simulink model "OnlyCurrent"  (R2025b)
settings: Solver=VariableStepAuto  StartTime=0.0  StopTime=0.3  MaxStep=1/20e3/100  RelTol=1e-3
InitFcn:
  | fs = 20e3;
  | Ts = 1/fs;
  | I2B = 10;
  | UB = 20;
  | freq0 = 50;
  | freqc = 5;
  | w0 = 2*pi / (1/freq0);
  | wc = 2*pi / (1/freqc);
  | I2_Kp = 3.023;
  | I2_Kr = 16.36;
  | UDC = 48;
  | Ic_Kd = 11.55;
libraries: ee_lib x26, nesl_utility x21, fl_lib x18, simulink x1
settings Model: Creator=GoodUser  LastModifiedBy=GoodUser

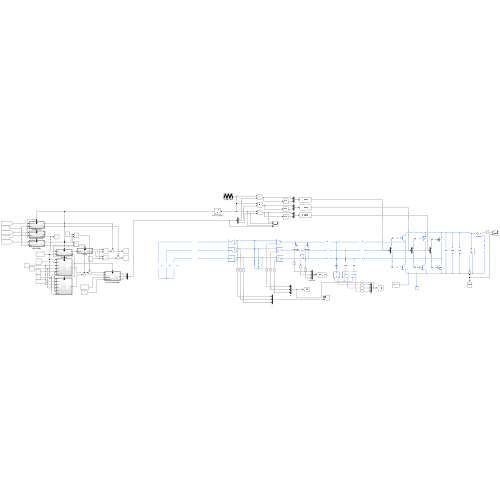
[thumbnail: Simulink's stored preview of the top-level diagram]
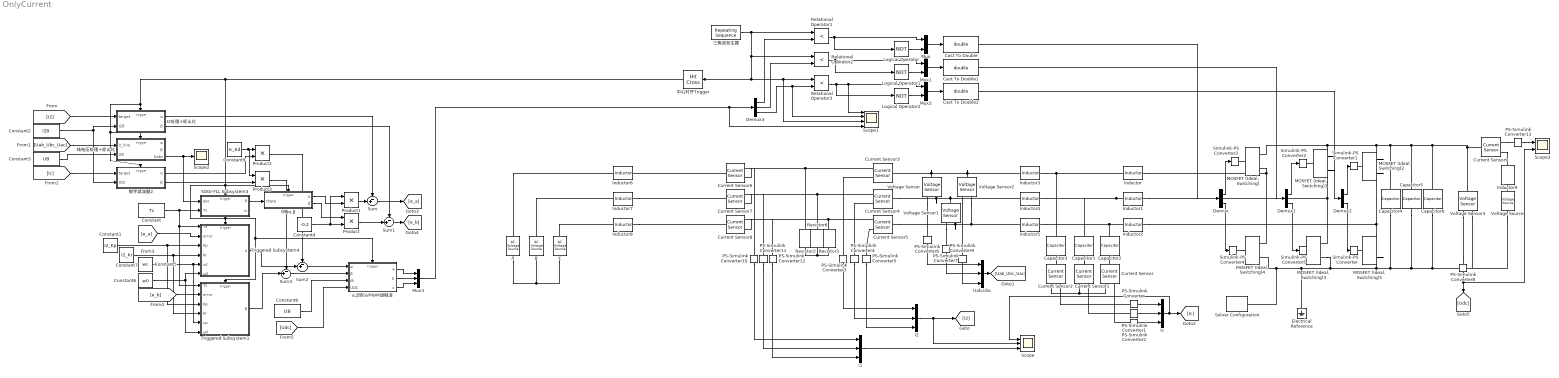
== system OnlyCurrent ==
  A : fl_lib/Electrical/Electrical Sources/AC Voltage Source  amp=20 V  shift=0 deg  frequency=50 Hz
  B : fl_lib/Electrical/Electrical Sources/AC Voltage Source  amp=20 V  shift=-120 deg  frequency=50 Hz
  C : fl_lib/Electrical/Electrical Sources/AC Voltage Source  amp=20 V  shift=120 deg  frequency=50 Hz
  Capacitor1 : ee_lib/Passive/Capacitor  cap_option=ee.enum.passive.capacitor.capOption.const  c=18e-6 F  Cvec=[1e-05, 1e-06] F  Vvec=[0, 10] V  CV_table_symmetry=ee.enum.passive.capacitor.tableSymmetry.yes  f_vec=[1, 10] kHz  DFext_vec=[.8, 1.2]  enable_C_tol=ee.enum.toleranceApplication.none  averaging_period=0 s  C_tol=5  tol_distribution=ee.enum.toleranceDistribution.uniform  nSigma=4  r=8e-3 Ohm  g=0 1/Ohm  enable_operating_limits=ee.enum.enable.no  operating_limit_action=ee.enum.passive.reportOpLim.warn  max_working_voltage_range=[-25, 25] V  power_rating=1 W  maxTemperature=85 degC  thermalEnable=false  thermalMass=1 J/K  i_specify=off  i_priority=None  i=0 A  i_nominal_specify=off  i_nominal_value=1  i_nominal_unit=A  v_specify=off  v_priority=None  v=0 V  v_nominal_specify=off  v_nominal_value=1  v_nominal_unit=V  vc_specify=off  vc_priority=High  vc=0 V  vc_nominal_specify=off  vc_nominal_value=1  vc_nominal_unit=V  T_specify=off  T_priority=None  T=298.15 K  T_nominal_specify=off  T_nominal_value=1  T_nominal_unit=K
  Capacitor2 : ee_lib/Passive/Capacitor  cap_option=ee.enum.passive.capacitor.capOption.const  c=18e-6 F  Cvec=[1e-05, 1e-06] F  Vvec=[0, 10] V  CV_table_symmetry=ee.enum.passive.capacitor.tableSymmetry.yes  f_vec=[1, 10] kHz  DFext_vec=[.8, 1.2]  enable_C_tol=ee.enum.toleranceApplication.none  averaging_period=0 s  C_tol=5  tol_distribution=ee.enum.toleranceDistribution.uniform  nSigma=4  r=8e-3 Ohm  g=0 1/Ohm  enable_operating_limits=ee.enum.enable.no  operating_limit_action=ee.enum.passive.reportOpLim.warn  max_working_voltage_range=[-25, 25] V  power_rating=1 W  maxTemperature=85 degC  thermalEnable=false  thermalMass=1 J/K  i_specify=off  i_priority=None  i=0 A  i_nominal_specify=off  i_nominal_value=1  i_nominal_unit=A  v_specify=off  v_priority=None  v=0 V  v_nominal_specify=off  v_nominal_value=1  v_nominal_unit=V  vc_specify=off  vc_priority=High  vc=0 V  vc_nominal_specify=off  vc_nominal_value=1  vc_nominal_unit=V  T_specify=off  T_priority=None  T=298.15 K  T_nominal_specify=off  T_nominal_value=1  T_nominal_unit=K
  Capacitor3 : ee_lib/Passive/Capacitor  cap_option=ee.enum.passive.capacitor.capOption.const  c=18e-6 F  Cvec=[1e-05, 1e-06] F  Vvec=[0, 10] V  CV_table_symmetry=ee.enum.passive.capacitor.tableSymmetry.yes  f_vec=[1, 10] kHz  DFext_vec=[.8, 1.2]  enable_C_tol=ee.enum.toleranceApplication.none  averaging_period=0 s  C_tol=5  tol_distribution=ee.enum.toleranceDistribution.uniform  nSigma=4  r=8e-3 Ohm  g=0 1/Ohm  enable_operating_limits=ee.enum.enable.no  operating_limit_action=ee.enum.passive.reportOpLim.warn  max_working_voltage_range=[-25, 25] V  power_rating=1 W  maxTemperature=85 degC  thermalEnable=false  thermalMass=1 J/K  i_specify=off  i_priority=None  i=0 A  i_nominal_specify=off  i_nominal_value=1  i_nominal_unit=A  v_specify=off  v_priority=None  v=0 V  v_nominal_specify=off  v_nominal_value=1  v_nominal_unit=V  vc_specify=off  vc_priority=High  vc=0 V  vc_nominal_specify=off  vc_nominal_value=1  vc_nominal_unit=V  T_specify=off  T_priority=None  T=298.15 K  T_nominal_specify=off  T_nominal_value=1  T_nominal_unit=K
  Capacitor4 : ee_lib/Passive/Capacitor  cap_option=ee.enum.passive.capacitor.capOption.const  c=1000e-6 F  Cvec=[1e-05, 1e-06] F  Vvec=[0, 10] V  CV_table_symmetry=ee.enum.passive.capacitor.tableSymmetry.yes  f_vec=[1, 10] kHz  DFext_vec=[.8, 1.2]  enable_C_tol=ee.enum.toleranceApplication.none  averaging_period=0 s  C_tol=5  tol_distribution=ee.enum.toleranceDistribution.uniform  nSigma=4  r=200e-3 Ohm  g=0 1/Ohm  enable_operating_limits=ee.enum.enable.no  operating_limit_action=ee.enum.passive.reportOpLim.warn  max_working_voltage_range=[-25, 25] V  power_rating=1 W  maxTemperature=85 degC  thermalEnable=false  thermalMass=1 J/K  i_specify=off  i_priority=None  i=0 A  i_nominal_specify=off  i_nominal_value=1  i_nominal_unit=A  v_specify=off  v_priority=None  v=0 V  v_nominal_specify=off  v_nominal_value=1  v_nominal_unit=V  vc_specify=off  vc_priority=High  vc=0 V  vc_nominal_specify=off  vc_nominal_value=1  vc_nominal_unit=V  T_specify=off  T_priority=None  T=298.15 K  T_nominal_specify=off  T_nominal_value=1  T_nominal_unit=K
  Capacitor5 : ee_lib/Passive/Capacitor  cap_option=ee.enum.passive.capacitor.capOption.const  c=1000e-6 F  Cvec=[1e-05, 1e-06] F  Vvec=[0, 10] V  CV_table_symmetry=ee.enum.passive.capacitor.tableSymmetry.yes  f_vec=[1, 10] kHz  DFext_vec=[.8, 1.2]  enable_C_tol=ee.enum.toleranceApplication.none  averaging_period=0 s  C_tol=5  tol_distribution=ee.enum.toleranceDistribution.uniform  nSigma=4  r=200e-3 Ohm  g=0 1/Ohm  enable_operating_limits=ee.enum.enable.no  operating_limit_action=ee.enum.passive.reportOpLim.warn  max_working_voltage_range=[-25, 25] V  power_rating=1 W  maxTemperature=85 degC  thermalEnable=false  thermalMass=1 J/K  i_specify=off  i_priority=None  i=0 A  i_nominal_specify=off  i_nominal_value=1  i_nominal_unit=A  v_specify=off  v_priority=None  v=0 V  v_nominal_specify=off  v_nominal_value=1  v_nominal_unit=V  vc_specify=off  vc_priority=High  vc=0 V  vc_nominal_specify=off  vc_nominal_value=1  vc_nominal_unit=V  T_specify=off  T_priority=None  T=298.15 K  T_nominal_specify=off  T_nominal_value=1  T_nominal_unit=K
  Capacitor6 : ee_lib/Passive/Capacitor  cap_option=ee.enum.passive.capacitor.capOption.const  c=1000e-6 F  Cvec=[1e-05, 1e-06] F  Vvec=[0, 10] V  CV_table_symmetry=ee.enum.passive.capacitor.tableSymmetry.yes  f_vec=[1, 10] kHz  DFext_vec=[.8, 1.2]  enable_C_tol=ee.enum.toleranceApplication.none  averaging_period=0 s  C_tol=5  tol_distribution=ee.enum.toleranceDistribution.uniform  nSigma=4  r=200e-3 Ohm  g=0 1/Ohm  enable_operating_limits=ee.enum.enable.no  operating_limit_action=ee.enum.passive.reportOpLim.warn  max_working_voltage_range=[-25, 25] V  power_rating=1 W  maxTemperature=85 degC  thermalEnable=false  thermalMass=1 J/K  i_specify=off  i_priority=None  i=0 A  i_nominal_specify=off  i_nominal_value=1  i_nominal_unit=A  v_specify=off  v_priority=None  v=0 V  v_nominal_specify=off  v_nominal_value=1  v_nominal_unit=V  vc_specify=off  vc_priority=High  vc=0 V  vc_nominal_specify=off  vc_nominal_value=1  vc_nominal_unit=V  T_specify=off  T_priority=None  T=298.15 K  T_nominal_specify=off  T_nominal_value=1  T_nominal_unit=K
  Cast To Double : DataTypeConversion  OutDataTypeStr=double  SaturateOnIntegerOverflow=off  RndMeth=Floor
  Cast To Double1 : DataTypeConversion  OutDataTypeStr=double  SaturateOnIntegerOverflow=off  RndMeth=Floor
  Cast To Double2 : DataTypeConversion  OutDataTypeStr=double  SaturateOnIntegerOverflow=off  RndMeth=Floor
  Constant : Constant  Value=Ts
  Constant1 : Constant  Value=I2_Kp
  Constant2 : Constant  Value=I2B
  Constant3 : Constant  Value=UB
  Constant4 : Constant  Value=-0.2
  Constant5 : Constant  Value=wc
  Constant6 : Constant  Value=w0
  Constant7 : Constant  Value=I2_Kr
  Constant8 : Constant  Value=I2B
  Constant9 : Constant  Value=Ic_Kd
  Current Sensor{,1..9} (10 alike) : fl_lib/Electrical/Electrical Sensors/Current Sensor
  Demux : Demux  Outputs=2
  Demux1 : Demux  Outputs=2
  Demux2 : Demux  Outputs=2
  Demux3 : Demux  Outputs=3
  Electrical Reference : fl_lib/Electrical/Electrical Elements/Electrical Reference
  I1 : Mux  Inputs=3
  I2 : Mux  Inputs=3
  I2处理+标幺化 : Subsystem  TreatAsAtomicUnit=on
  Ic : Mux  Inputs=3
  Inductor : ee_lib/Passive/Inductor  l=400e-6 H  enable_L_tol=ee.enum.toleranceApplication.none  L_tol=20  tol_distribution=ee.enum.toleranceDistribution.uniform  nSigma=4  r=30e-3 Ohm  g=1e-9 1/Ohm  enable_operating_limits=ee.enum.enable.no  operating_limit_action=ee.enum.passive.reportOpLim.warn  max_working_current=1 A  power_rating=1 W  i_L_specify=off  i_L_priority=High  i_L=0 A  i_L_nominal_specify=off  i_L_nominal_value=1  i_L_nominal_unit=A
  Inductor1 : ee_lib/Passive/Inductor  l=400e-6 H  enable_L_tol=ee.enum.toleranceApplication.none  L_tol=20  tol_distribution=ee.enum.toleranceDistribution.uniform  nSigma=4  r=30e-3 Ohm  g=1e-9 1/Ohm  enable_operating_limits=ee.enum.enable.no  operating_limit_action=ee.enum.passive.reportOpLim.warn  max_working_current=1 A  power_rating=1 W  i_L_specify=off  i_L_priority=High  i_L=0 A  i_L_nominal_specify=off  i_L_nominal_value=1  i_L_nominal_unit=A
  Inductor2 : ee_lib/Passive/Inductor  l=400e-6 H  enable_L_tol=ee.enum.toleranceApplication.none  L_tol=20  tol_distribution=ee.enum.toleranceDistribution.uniform  nSigma=4  r=30e-3 Ohm  g=1e-9 1/Ohm  enable_operating_limits=ee.enum.enable.no  operating_limit_action=ee.enum.passive.reportOpLim.warn  max_working_current=1 A  power_rating=1 W  i_L_specify=off  i_L_priority=High  i_L=0 A  i_L_nominal_specify=off  i_L_nominal_value=1  i_L_nominal_unit=A
  Inductor{3..8} (6 alike) : ee_lib/Passive/Inductor  l=200e-6 H  enable_L_tol=ee.enum.toleranceApplication.none  L_tol=20  tol_distribution=ee.enum.toleranceDistribution.uniform  nSigma=4  r=15e-3 Ohm  g=1e-9 1/Ohm  enable_operating_limits=ee.enum.enable.no  operating_limit_action=ee.enum.passive.reportOpLim.warn  max_working_current=1 A  power_rating=1 W  i_L_specify=off  i_L_priority=High  i_L=0 A  i_L_nominal_specify=off  i_L_nominal_value=1  i_L_nominal_unit=A
  Inductor9 : ee_lib/Passive/Inductor  l=100e-9 H  enable_L_tol=ee.enum.toleranceApplication.none  L_tol=20  tol_distribution=ee.enum.toleranceDistribution.uniform  nSigma=4  r=10e-3 Ohm  g=1e-9 1/Ohm  enable_operating_limits=ee.enum.enable.no  operating_limit_action=ee.enum.passive.reportOpLim.warn  max_working_current=1 A  power_rating=1 W  i_L_specify=off  i_L_priority=High  i_L=0 A  i_L_nominal_specify=off  i_L_nominal_value=1  i_L_nominal_unit=A
  Logical Operator : Logic  Operator=NOT  AllPortsSameDT=off  OutDataTypeStr=boolean
  Logical Operator1 : Logic  Operator=NOT  AllPortsSameDT=off  OutDataTypeStr=boolean
  Logical Operator2 : Logic  Operator=NOT  AllPortsSameDT=off  OutDataTypeStr=boolean
  MOSFET (Ideal, Switching){,1..5} (6 alike) : ee_lib/Semiconductors & Converters/MOSFET (Ideal, Switching)  port_option=ee.enum.controlport.ps  Rds=0.01 Ohm  Goff=1e-6 1/Ohm  Vth=0.9 V  diode_param=ee.enum.semiconductors.protectionDiode.nodynamics  diode_Vf=0.8 V  diode_Ron=0.001 Ohm  diode_Goff=1e-5 1/Ohm  diode_C=50e-9 F  diode_iRM=-235 A  diode_iF=300 A  diode_idot=-50 A/us  diode_trr_param=ee.enum.converters.diodeReverseParam.trr_factor  diode_trr_factor=3  diode_trr=15 us  diode_Qrr=1500 s*uA  ids_specify=off  ids_priority=None  ids=0 A  ids_nominal_specify=off  ids_nominal_value=1  ids_nominal_unit=A  vds_specify=off  vds_priority=None  vds=0 V  vds_nominal_specify=off  vds_nominal_value=1  vds_nominal_unit=V  vgs_specify=off  vgs_priority=None  vgs=0 V  vgs_nominal_specify=off  vgs_nominal_value=1  vgs_nominal_unit=V  thermal_loss_option=ee.enum.converters.thermalLossOption.constantvalues  Von_data=[0, 1.8, 3.2, 6, 10, 16; 0, 2, 5.5, 9.5, 15, 25] V  Tj=[298.15, 448.15] K  Iout_data=[0, 20, 40, 60, 80, 100] A  Eon_data=[0, 55.04, 124.57, 235.53, 362.12; 0, 71.25, 161.25, 304.88, 468.75] * 1e-6 J  Eoff_data=[0, 18, 30, 56.1, 76.5; 0, 22.5, 37.5, 70.13, 95.63] * 1e-6 J  Eon_data_3D=[zeros(2, 5, 3)] J  Eoff_data_3D=[zeros(2, 5, 3)] J  Tj_loss=[298.15, 448.15] K  Iout_data_loss=[0, 10, 20, 30, 40] A  tabulateWithVds=false  Vds_loss=[0, 150, 300] V  Eon_scalar=22.86e-3 J  Eoff_scalar=17.14e-3 J  Voff=300 V  Iout_scalar=600 A  useCurrentFromPreviousCycle=false  useVoltageFromPreviousCycle=false  diodeModelType=ee.enum.converters.diodeModelType.pwl  diodeTableType=ee.enum.diode.tableType.IfMat  diode_ReverseIVType=ee.enum.diode.diodeReverseIV.constant  diode_IfMat=[.07, .12, .19, 1.75, 4.24, 7.32, 11.2; .16, .3, .72, 2.14, 4.02, 6.35, 9.12] A  diode_VfMat=[.9, 1.15, 1.25, 1.5, 1.75, 2.17, 2.6, 2.85; .58, .68, .75, 1.1, 1.38, 1.77, 2.27, 2.7] V  diode_TjVec=[25, 125] degC  diode_VfVec=[.5, .7, .9, 1.3, 1.7, 2.1, 2.5] V  diode_IfVec=[.1, .2, .5, 1, 2, 4, 7, 10] A  diode_IrMat=[1e-06, 2e-06, 5e-06, 1e-05, 2.5e-05, 5e-05, .0001; 2e-06, 5e-06, 1e-05, 4e-05, 8e-05, .0002, .0005] A  diode_VrMat=[10, 100, 200, 250, 300, 325, 350; 10, 70, 160, 220, 270, 300, 320] V  diode_VrVec=[10, 20, 40, 50, 70, 80, 100] V  diode_IrVec=[1e-06, 2e-06, 5e-06, 1e-05, 2e-05, 5e-05, .0001] A  diode_Vr=-600 V  diode_Ls=150 nH  diode_Erec=0.03 J  diode_rec_loss_model=ee.enum.diode.reverseRecoveryModel.fixed  diode_ErecVal=0 J  diode_scaleWithIandV=true  diode_ErecMat=zeros(2, 3) J  diode_TjrecVec=[298.15, 398.15] K  diode_IfrecVec=[.1, 1, 10] A  diode_IrecVal=10 A  diode_VrecVal=10 V  diode_tFilter=1 / 1000 / 100 s  separateThermalPortForDiode=false  thermal_network_parameterization=ee.enum.thermalNetworkTopology.external  Rth=[.03, .2] K/W  Rth_Cauer=[.03, .1, .2] K/W  Rth_Foster=[.08, .14, .22, .16] K/W  thermal_mass_parameterization=ee.enum.thermalNetwork.timeconstant  thermal_mass=[3, 25] J/K  thermal_mass_Cauer=[3, 10, 25] J/K  thermal_mass_Foster=[.001, .005, .05, .5] J/K  thermal_time_constant=[.1, 5] s  thermal_time_constant_Cauer=[.1, 1, 5] s  thermal_time_constant_Foster=[7e-05, .0007, .01, .08] s  thermal_mass_initial_temperatures=[25, 25] degC  thermal_mass_initial_temperatures_Cauer=[25, 25, 25] degC  junction_thermal_mass=0.1 J/K  Tvec_initial_Foster=[25, 25, 25, 25] degC  RthDiode=[.03, .2] K/W  RthCauerDiode=[.03, .1, .2] K/W  RthFosterDiode=[.03, .2] K/W  thermalMassDiode=[3, 25] J/K  thermalMassCauerDiode=[3, 10, 25] J/K  thermalMassFosterDiode=[33, 50] J/K  thermalTauDiode=[.1, 5] s  thermalTauCauerDiode=[.1, 1, 5] s  thermalTauFosterDiode=[1, 10] s  thermalMassInitTempDiode=[25, 25] degC  thermalMassInitTempCauerDiode=[25, 25, 25] degC  junctionthermalMassDiode=0.1 J/K  TVecInitialFosterDiode=[25, 25, 25, 25] degC  no_thermal_network=0  mosfet_junction_temperature_specify=off  mosfet_junction_temperature_priority=None  mosfet_junction_temperature=25 degC  mosfet_junction_temperature_nominal_specify=off  mosfet_junction_temperature_nominal_value=1  mosfet_junction_temperature_nominal_unit=degC  diode_junction_temperature_specify=off  diode_junction_temperature_priority=None  diode_junction_temperature=25 degC  diode_junction_temperature_nominal_specify=off  diode_junction_temperature_nominal_value=1  diode_junction_temperature_nominal_unit=degC  Qj_specify=off  Qj_priority=None  Qj=0 W  Qj_nominal_specify=off  Qj_nominal_value=1  Qj_nominal_unit=W  accumulatedSwitchingLosses_specify=off  accumulatedSwitchingLosses_priority=None  accumulatedSwitchingLosses=0 J
  Mux : Mux  Inputs=2
  Mux1 : Mux  Inputs=2
  Mux2 : Mux  Inputs=2
  Mux3 : Mux  Inputs=3
  PS-Simulink Converter{,1..13} (14 alike) : nesl_utility/PS-Simulink Converter  PhysicalDomain=network_engine_domain  SubClassName=ps_output  LeftPortType=input  RightPortType=output  PseudoPeriodic=off  Frequencies=[]  VectorFormat=inherit  Unit=inherit  AffineConversion=off
  Product{,1..3} (4 alike) : Product
  Relational Operator1 : RelationalOperator  Operator=<  OutDataTypeStr=boolean  RndMeth=Simplest  InputSameDT=off
  Relational Operator2 : RelationalOperator  Operator=<  OutDataTypeStr=boolean  RndMeth=Simplest  InputSameDT=off
  Relational Operator3 : RelationalOperator  Operator=<  OutDataTypeStr=boolean  RndMeth=Simplest  InputSameDT=off
  Resistor2 : ee_lib/Passive/Resistor  R=100 Ohm  enable_R_tol=ee.enum.toleranceApplication.none  R_tol=5  tol_distribution=ee.enum.toleranceDistribution.uniform  nSigma=4  enable_operating_limits=ee.enum.enable.no  operating_limit_action=ee.enum.passive.reportOpLim.warn  power_rating=1 W  max_working_voltage=100 V  noise_mode=ee.enum.sources.noise.Disabled  Tdevice=25 degC  sample_time=1e-3 s  repeatability=ee.enum.ic.repeatability.notRepeatable  user_seed=0  auto_seed=1826474873  power_derating_T1=70 degC  power_derating_T2=155 degC  operating_temperature_range_vec=[-50, 150] degC  alpha=3.93e-3 1/K  Tmeas=25 degC  thermal_mass=100 J/K  temperature_specify=off  temperature_priority=High  temperature=298.15 K  temperature_nominal_specify=off  temperature_nominal_value=1  temperature_nominal_unit=K
  Resistor3 : ee_lib/Passive/Resistor  R=100 Ohm  enable_R_tol=ee.enum.toleranceApplication.none  R_tol=5  tol_distribution=ee.enum.toleranceDistribution.uniform  nSigma=4  enable_operating_limits=ee.enum.enable.no  operating_limit_action=ee.enum.passive.reportOpLim.warn  power_rating=1 W  max_working_voltage=100 V  noise_mode=ee.enum.sources.noise.Disabled  Tdevice=25 degC  sample_time=1e-3 s  repeatability=ee.enum.ic.repeatability.notRepeatable  user_seed=0  auto_seed=693571696  power_derating_T1=70 degC  power_derating_T2=155 degC  operating_temperature_range_vec=[-50, 150] degC  alpha=3.93e-3 1/K  Tmeas=25 degC  thermal_mass=100 J/K  temperature_specify=off  temperature_priority=High  temperature=298.15 K  temperature_nominal_specify=off  temperature_nominal_value=1  temperature_nominal_unit=K
  Resistor6 : ee_lib/Passive/Resistor  R=100 Ohm  enable_R_tol=ee.enum.toleranceApplication.none  R_tol=5  tol_distribution=ee.enum.toleranceDistribution.uniform  nSigma=4  enable_operating_limits=ee.enum.enable.no  operating_limit_action=ee.enum.passive.reportOpLim.warn  power_rating=1 W  max_working_voltage=100 V  noise_mode=ee.enum.sources.noise.Disabled  Tdevice=25 degC  sample_time=1e-3 s  repeatability=ee.enum.ic.repeatability.notRepeatable  user_seed=0  auto_seed=1343117392  power_derating_T1=70 degC  power_derating_T2=155 degC  operating_temperature_range_vec=[-50, 150] degC  alpha=3.93e-3 1/K  Tmeas=25 degC  thermal_mass=100 J/K  temperature_specify=off  temperature_priority=High  temperature=298.15 K  temperature_nominal_specify=off  temperature_nominal_value=1  temperature_nominal_unit=K
  SOGI-FLL Subsystem3 : Subsystem  TreatAsAtomicUnit=on
  Scope : Scope  NumInputPorts=3
      settings: ActiveDisplayYMinimum=-4.8299942276890091  ActiveDisplayYMaximum=4.7601258533296331
  Scope1 : Scope  NumInputPorts=4
      settings: ActiveDisplayYMinimum=-0.12499999999999997  ActiveDisplayYMaximum=1.125
  Scope2 : Scope
      settings: ActiveDisplayYMinimum=10.733460497703403  ActiveDisplayYMaximum=15.152374451772815  DataLoggingVariableName=ScopeData2
  Scope3 : Scope  NumInputPorts=2
      settings: ActiveDisplayYMinimum=47.899284509221786  ActiveDisplayYMaximum=48.164122496405994  DataLoggingVariableName=ScopeData3
  Simulink-PS Converter{,1..5} (6 alike) : nesl_utility/Simulink-PS Converter  PhysicalDomain=network_engine_domain  SubClassName=ps_input  LeftPortType=input  RightPortType=output  PseudoPeriodic=off  Frequencies=[]  NoiseDistribution=none  NoiseParameters=[]  Unit=1  AffineConversion=off  FilteringAndDerivatives=provide  SimscapeFilterOrder=1  InputFilterTimeConstant=0.001  UdotUserProvided=0
  Solver Configuration : nesl_utility/Solver Configuration  PhysicalDomain=network_engine_domain  SubClassName=solver  LeftPortType=input  RightPortType=generic  Tones=[]  Harmonics=[]  SimulateNoise=off  Profile=off  UseLocalSampling=off  EnableSwitchedLinearOptims=on  FrequencyDomain=off  UseCCode=off  RelTol=0.001  AbsTol=0.001  MinStep=1e-09  ToWorkspace=off  RevertToSquareIcSolve=off  NumHomotopyIterations=100  PhasorMode=off  PhasorModeNumHarmonics=1  ConsistencySolver=NEWTON_XTOL_AFTER_FTOL  IndexReductionMethod=DerivativeReplacement  DoDC=off  ResidualTolerance=1e-09  ConsistencyTolSource=GLOBAL  ConsistencyAbsTol=0.001  ConsistencyRelTol=0.001  ConsistencyTolFactor=0.001  UseLocalSolver=on  LocalSolverChoice=NE_BACKWARD_EULER_ADVANCER  ResolveIndetEquations=on  FunctionEvalNumThread=1  LocalSolverSampleTime=1/20e3/100  DoFixedCost=off  MaxNonlinIter=3  MaxModeIter=2  ComputeImpulses=off  ImpulseIterations=2  LinearAlgebra=auto  LinearAlgebraNumThread=0  EquationFormulation=NE_TIME_EF  DelaysMemoryBudget=1024  AutomaticFiltering=on  FilteringTimeConstant=0.001  PartitionStorageMethod=AS_NEEDED  PartitionMemoryBudget=1024  PartitionMethod=ROBUST  MultibodyUseLocalSolver=off  MultibodyLocalSolverChoice=ODE1  MultibodyLocalSolverSampleTime=0.001
  Sum{,1..3} (4 alike) : Sum  Inputs=-+|
  Triggered Subsystem1 : Subsystem  TreatAsAtomicUnit=on
  Triggered Subsystem4 : Subsystem  TreatAsAtomicUnit=on
  Uab,Ubc : Mux  Inputs=3
  Voltage Sensor{,1..3} (4 alike) : fl_lib/Electrical/Electrical Sensors/Voltage Sensor
  Voltage Source : ee_lib/Sources/Voltage Source  dc_voltage=48 V  ac_voltage=0 V  ac_shift=0 rad  ac_frequency=60 Hz  noise_mode=ee.enum.sources.noise.Disabled  PSD=0 V^2/Hz  sample_time=1e-3 s  repeatability=ee.enum.sources.repeatability.NotRepeatable  user_seed=0  auto_seed=545404223  i_specify=off  i_priority=None  i=0 A  i_nominal_specify=off  i_nominal_value=1  i_nominal_unit=A  v_specify=off  v_priority=None  v=0 V  v_nominal_specify=off  v_nominal_value=1  v_nominal_unit=V
  α,β转SVPWM调制波 : Subsystem  TreatAsAtomicUnit=on
  θ转α,β : Subsystem  TreatAsAtomicUnit=on
  三角波发生器 : simulink/Sources/Repeating Sequence  rep_seq_t=[0 Ts/2 Ts]  rep_seq_y=[0 1 0]
  中心对齐Trigger : HitCross  HitCrossingOffset=0.00  HitCrossingDirection=rising
  数字滤波器2 : Subsystem  TreatAsAtomicUnit=on
  线电压处理+标幺化 : Subsystem  TreatAsAtomicUnit=on
  wires:
  PS-Simulink Converter/1 -> Ic/1
  PS-Simulink Converter1/1 -> Ic/2
  PS-Simulink Converter2/1 -> Ic/3
  PS-Simulink Converter3/1 -> I2/1
  PS-Simulink Converter4/1 -> I2/2
  PS-Simulink Converter5/1 -> I2/3
  PS-Simulink Converter7/1 -> Uab,Ubc/2
  PS-Simulink Converter6/1 -> Uab,Ubc/1
  Demux3/1 -> Relational Operator1/2
  Relational Operator2/1 -> Mux1/1, Logical Operator1/1
  Demux3/2 -> Relational Operator2/2
  三角波发生器/1 -> Relational Operator1/1, 中心对齐Trigger/1, Scope1/3, Relational Operator3/1, Relational Operator2/1
  Demux3/3 -> Scope1/2, Relational Operator3/2
  Mux/1 -> Cast To Double/1
  Mux1/1 -> Cast To Double1/1
  Ic/1 -> Scope/1, [Ic]
  Logical Operator1/1 -> Mux1/2
  Logical Operator/1 -> Mux/2
  Logical Operator2/1 -> Mux2/2
  Mux2/1 -> Cast To Double2/1
  Relational Operator3/1 -> Logical Operator2/1, Scope1/1, Mux2/1
  Relational Operator1/1 -> Logical Operator/1, Mux/1
  Demux1/1 -> Simulink-PS Converter2/1
  Demux1/2 -> Simulink-PS Converter5/1
  Demux/1 -> Simulink-PS Converter3/1
  Demux/2 -> Simulink-PS Converter4/1
  Demux2/1 -> Simulink-PS Converter1/1
  Demux2/2 -> Simulink-PS Converter/1
  Cast To Double/1 -> Demux/1
  Cast To Double1/1 -> Demux1/1
  Cast To Double2/1 -> Demux2/1
  中心对齐Trigger/1 -> 线电压处理+标幺化/Trigger, 数字滤波器2/Trigger, I2处理+标幺化/Trigger, SOGI-FLL Subsystem3/Trigger, Triggered Subsystem4/Trigger, α,β转SVPWM调制波/Trigger, Triggered Subsystem1/Trigger, θ转α,β/Trigger
  I2/1 -> Scope/2, [I2]
  Uab,Ubc/1 -> [Uab_Ubc_Uac]
  [I2] -> I2处理+标幺化/1(target)
  [Uab_Ubc_Uac] -> 线电压处理+标幺化/1(U_line)
  线电压处理+标幺化/3(Uabc) -> SOGI-FLL Subsystem3/1(abc), Scope2/1
  PS-Simulink Converter9/1 -> Uab,Ubc/3
  Constant/1 -> SOGI-FLL Subsystem3/2(Ts), Triggered Subsystem1/1(Ts), Triggered Subsystem4/1(Ts)
  Mux3/1 -> Scope1/4, Demux3/1
  Constant2/1 -> 数字滤波器2/2(ICB), I2处理+标幺化/2(I2B)
  Constant3/1 -> 线电压处理+标幺化/2(UB)
  SOGI-FLL Subsystem3/1(θ) -> θ转α,β/1(theta)
  [Ic] -> 数字滤波器2/1(target)
  Product1/1 -> Sum/2
  Constant4/1 -> Product1/1, Product/2
  Product/1 -> Sum1/2
  Sum/1 -> [e_a]
  Sum1/1 -> [e_b]
  [e_a] -> Triggered Subsystem4/2(error)
  Constant5/1 -> Triggered Subsystem1/5(ωc), Triggered Subsystem4/5(ωc)
  Constant6/1 -> Triggered Subsystem4/6(ω0), Triggered Subsystem1/6(ω0)
  [e_b] -> Triggered Subsystem1/2(error)
  Triggered Subsystem4/1(α) -> Sum2/2
  α,β转SVPWM调制波/1(a) -> Mux3/1
  α,β转SVPWM调制波/2(b) -> Mux3/2
  α,β转SVPWM调制波/3(c) -> Mux3/3
  Constant8/1 -> α,β转SVPWM调制波/3(IB)
  PS-Simulink Converter8/1 -> Scope3/2, [Udc]
  [Udc] -> α,β转SVPWM调制波/4(UDC)
  Constant7/1 -> Triggered Subsystem4/4(Kr), Triggered Subsystem1/4(Kr)
  Constant1/1 -> Triggered Subsystem4/3(Kp), Triggered Subsystem1/3(Kp)
  PS-Simulink Converter10/1 -> I1/1
  PS-Simulink Converter11/1 -> I1/2
  PS-Simulink Converter12/1 -> I1/3
  I1/1 -> Scope/3
  数字滤波器2/1(α) -> Product2/2
  I2处理+标幺化/1(α) -> Sum/1
  Constant9/1 -> Product3/1, Product2/1
  数字滤波器2/2(β) -> Product3/2
  I2处理+标幺化/2(β) -> Sum1/1
  Sum2/1 -> α,β转SVPWM调制波/1(α)
  Sum3/1 -> α,β转SVPWM调制波/2(β)
  Triggered Subsystem1/1(β) -> Sum3/2
  Product2/1 -> Sum2/1
  Product3/1 -> Sum3/1
  θ转α,β/2(β) -> Product/1
  θ转α,β/1(α) -> Product1/2
  PS-Simulink Converter13/1 -> Scope3/1
  connections:
  Capacitor6/RConn1 -- Voltage Source/RConn1 -- Voltage Sensor3/RConn2 -- Capacitor5/RConn1 -- Capacitor4/RConn1 -- "MOSFET (Ideal, Switching)5"/RConn2 -- "MOSFET (Ideal, Switching)3"/RConn2 -- Electrical Reference/LConn1 -- Solver Configuration/RConn1 -- "MOSFET (Ideal, Switching)4"/RConn2
  Voltage Sensor3/LConn1 -- Capacitor6/LConn1 -- Capacitor5/LConn1 -- Capacitor4/LConn1 -- "MOSFET (Ideal, Switching)"/RConn1 -- "MOSFET (Ideal, Switching)1"/RConn1 -- "MOSFET (Ideal, Switching)2"/RConn1 -- Current Sensor9/LConn1
  Inductor/LConn1 -- Capacitor3/LConn1 -- Inductor3/RConn1
  Inductor1/LConn1 -- Inductor4/RConn1 -- Capacitor1/LConn1
  Capacitor2/LConn1 -- Inductor5/RConn1 -- Inductor2/LConn1
  Current Sensor1/RConn2 -- Current Sensor/RConn2 -- Current Sensor2/RConn2
  Voltage Sensor2/LConn1 -- Inductor3/LConn1 -- Voltage Sensor/LConn1 -- Current Sensor3/LConn1
  Current Sensor/LConn1 -- Capacitor2/RConn1
  Capacitor1/RConn1 -- Current Sensor1/LConn1
  Capacitor3/RConn1 -- Current Sensor2/LConn1
  Current Sensor2/RConn1 -- PS-Simulink Converter/LConn1
  PS-Simulink Converter1/LConn1 -- Current Sensor1/RConn1
  PS-Simulink Converter2/LConn1 -- Current Sensor/RConn1
  Current Sensor4/LConn1 -- Voltage Sensor/RConn2 -- Inductor4/LConn1 -- Voltage Sensor1/LConn1
  Current Sensor5/LConn1 -- Inductor5/LConn1 -- Voltage Sensor2/RConn2 -- Voltage Sensor1/RConn2
  Current Sensor7/RConn2 -- Resistor6/LConn1 -- Current Sensor4/RConn2
  PS-Simulink Converter3/LConn1 -- Current Sensor3/RConn1
  Current Sensor4/RConn1 -- PS-Simulink Converter4/LConn1
  PS-Simulink Converter5/LConn1 -- Current Sensor5/RConn1
  Voltage Sensor/RConn1 -- PS-Simulink Converter6/LConn1
  Voltage Sensor1/RConn1 -- PS-Simulink Converter7/LConn1
  "MOSFET (Ideal, Switching)"/RConn2 -- Inductor/RConn1 -- "MOSFET (Ideal, Switching)4"/RConn1
  "MOSFET (Ideal, Switching)1"/RConn2 -- Inductor1/RConn1 -- "MOSFET (Ideal, Switching)3"/RConn1
  "MOSFET (Ideal, Switching)2"/RConn2 -- "MOSFET (Ideal, Switching)5"/RConn1 -- Inductor2/RConn1
  Simulink-PS Converter/RConn1 -- "MOSFET (Ideal, Switching)5"/LConn1
  Simulink-PS Converter1/RConn1 -- "MOSFET (Ideal, Switching)2"/LConn1
  Simulink-PS Converter3/RConn1 -- "MOSFET (Ideal, Switching)"/LConn1
  Simulink-PS Converter4/RConn1 -- "MOSFET (Ideal, Switching)4"/LConn1
  Simulink-PS Converter5/RConn1 -- "MOSFET (Ideal, Switching)3"/LConn1
  Voltage Sensor2/RConn1 -- PS-Simulink Converter9/LConn1
  C/RConn1 -- A/RConn1 -- B/RConn1
  Current Sensor6/RConn2 -- Resistor2/LConn1 -- Current Sensor3/RConn2
  Current Sensor8/RConn2 -- Resistor3/LConn1 -- Current Sensor5/RConn2
  Voltage Sensor3/RConn1 -- PS-Simulink Converter8/LConn1
  Current Sensor6/LConn1 -- Inductor6/RConn1
  Current Sensor6/RConn1 -- PS-Simulink Converter10/LConn1
  Current Sensor7/RConn1 -- PS-Simulink Converter11/LConn1
  Current Sensor8/RConn1 -- PS-Simulink Converter12/LConn1
  Resistor3/RConn1 -- Resistor2/RConn1 -- Resistor6/RConn1
  Simulink-PS Converter2/RConn1 -- "MOSFET (Ideal, Switching)1"/LConn1
  Inductor7/RConn1 -- Current Sensor7/LConn1
  Inductor8/RConn1 -- Current Sensor8/LConn1
  B/LConn1 -- Inductor7/LConn1
  A/LConn1 -- Inductor6/LConn1
  C/LConn1 -- Inductor8/LConn1
  Inductor9/RConn1 -- Voltage Source/LConn1
  Current Sensor9/RConn1 -- PS-Simulink Converter13/LConn1
  Current Sensor9/RConn2 -- Inductor9/LConn1

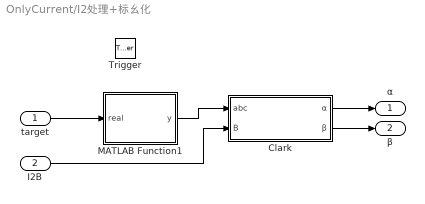
== system OnlyCurrent/I2处理+标幺化 ==
  target : Inport  LatchByDelayingOutsideSignal=on
  I2B : Inport  Port=2
  Trigger : TriggerPort  VariantControl=(inherit)
  Clark : Subsystem  TreatAsAtomicUnit=on
  MATLAB Function1 : MATLAB Function  TreatAsAtomicUnit=on
  α : Outport
  β : Outport  Port=2
  wires:
  target/1 -> MATLAB Function1/1(real)
  MATLAB Function1/1(y) -> Clark/1(abc)
  Clark/1(α) -> α/1
  Clark/2(β) -> β/1
  I2B/1 -> Clark/2(B)

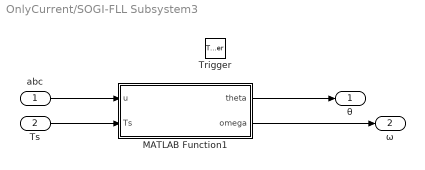
== system OnlyCurrent/SOGI-FLL Subsystem3 ==
  abc : Inport
  Ts : Inport  Port=2
  Trigger : TriggerPort  VariantControl=(inherit)
  MATLAB Function1 : MATLAB Function  TreatAsAtomicUnit=on
  θ : Outport
  ω : Outport  Port=2
  wires:
  MATLAB Function1/2(omega) -> ω/1
  abc/1 -> MATLAB Function1/1(u)
  MATLAB Function1/1(theta) -> θ/1
  Ts/1 -> MATLAB Function1/2(Ts)

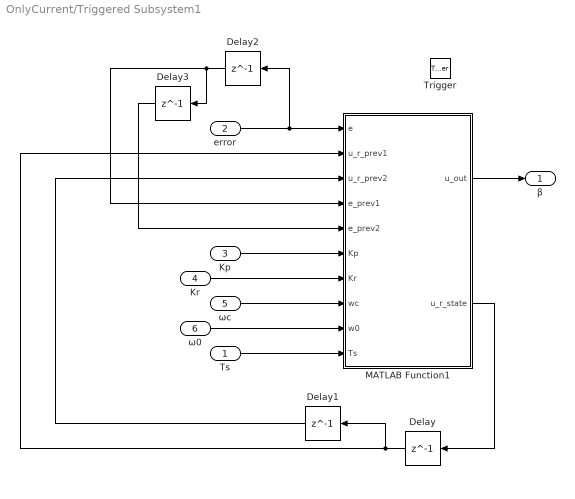
== system OnlyCurrent/Triggered Subsystem1 ==
  Ts : Inport
  error : Inport  Port=2
  Kp : Inport  Port=3
  Kr : Inport  Port=4
  ωc : Inport  Port=5
  ω0 : Inport  Port=6
  Trigger : TriggerPort  VariantControl=(inherit)
  Delay{,1..3} (4 alike) : Delay  DelayLength=1  InitialCondition=0
  MATLAB Function1 : MATLAB Function  TreatAsAtomicUnit=on
  β : Outport
  wires:
  Delay3/1 -> MATLAB Function1/5(e_prev2)
  Delay2/1 -> MATLAB Function1/4(e_prev1), Delay3/1
  error/1 -> MATLAB Function1/1(e), Delay2/1
  Delay1/1 -> MATLAB Function1/3(u_r_prev2)
  Delay/1 -> MATLAB Function1/2(u_r_prev1), Delay1/1
  MATLAB Function1/2(u_r_state) -> Delay/1
  Kp/1 -> MATLAB Function1/6(Kp)
  Kr/1 -> MATLAB Function1/7(Kr)
  ωc/1 -> MATLAB Function1/8(wc)
  ω0/1 -> MATLAB Function1/9(w0)
  Ts/1 -> MATLAB Function1/10(Ts)
  MATLAB Function1/1(u_out) -> β/1

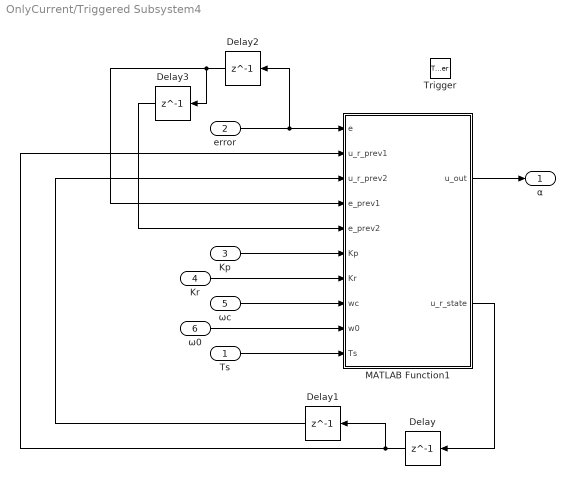
== system OnlyCurrent/Triggered Subsystem4 ==
  Ts : Inport
  error : Inport  Port=2
  Kp : Inport  Port=3
  Kr : Inport  Port=4
  ωc : Inport  Port=5
  ω0 : Inport  Port=6
  Trigger : TriggerPort  VariantControl=(inherit)
  Delay{,1..3} (4 alike) : Delay  DelayLength=1  InitialCondition=0
  MATLAB Function1 : MATLAB Function  TreatAsAtomicUnit=on
  α : Outport
  wires:
  MATLAB Function1/1(u_out) -> α/1
  Ts/1 -> MATLAB Function1/10(Ts)
  ω0/1 -> MATLAB Function1/9(w0)
  ωc/1 -> MATLAB Function1/8(wc)
  Kr/1 -> MATLAB Function1/7(Kr)
  Kp/1 -> MATLAB Function1/6(Kp)
  MATLAB Function1/2(u_r_state) -> Delay/1
  Delay/1 -> Delay1/1, MATLAB Function1/2(u_r_prev1)
  Delay1/1 -> MATLAB Function1/3(u_r_prev2)
  error/1 -> Delay2/1, MATLAB Function1/1(e)
  Delay2/1 -> Delay3/1, MATLAB Function1/4(e_prev1)
  Delay3/1 -> MATLAB Function1/5(e_prev2)

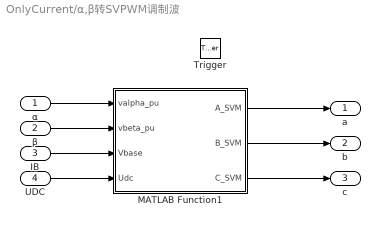
== system OnlyCurrent/α,β转SVPWM调制波 ==
  α : Inport
  β : Inport  Port=2
  IB : Inport  Port=3  LatchByDelayingOutsideSignal=on
  UDC : Inport  Port=4  LatchByDelayingOutsideSignal=on
  Trigger : TriggerPort  VariantControl=(inherit)
  MATLAB Function1 : MATLAB Function  TreatAsAtomicUnit=on
  a : Outport
  b : Outport  Port=2
  c : Outport  Port=3
  wires:
  MATLAB Function1/2(B_SVM) -> b/1
  α/1 -> MATLAB Function1/1(valpha_pu)
  MATLAB Function1/1(A_SVM) -> a/1
  MATLAB Function1/3(C_SVM) -> c/1
  β/1 -> MATLAB Function1/2(vbeta_pu)
  IB/1 -> MATLAB Function1/3(Vbase)
  UDC/1 -> MATLAB Function1/4(Udc)

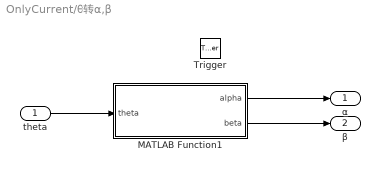
== system OnlyCurrent/θ转α,β ==
  theta : Inport
  Trigger : TriggerPort  VariantControl=(inherit)
  MATLAB Function1 : MATLAB Function  TreatAsAtomicUnit=on
  α : Outport
  β : Outport  Port=2
  wires:
  MATLAB Function1/1(alpha) -> α/1
  theta/1 -> MATLAB Function1/1(theta)
  MATLAB Function1/2(beta) -> β/1

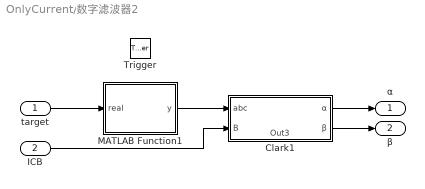
== system OnlyCurrent/数字滤波器2 ==
  target : Inport  LatchByDelayingOutsideSignal=on
  ICB : Inport  Port=2
  Trigger : TriggerPort  VariantControl=(inherit)
  Clark1 : Subsystem  TreatAsAtomicUnit=on
      settings: PortSchema="{\"entries\":[{\"content\":{\"sides\":[{\"content\":{\"connectorIds\":[\"In1\",\"In2\"]},\"type\":\"ConnectorPlacement.EquallySpacedRectSide\",\"uuid\":\"5266b147-56b7-4e2a-a13b-4b3ad7884dce\"},{\"content\":{\"connectorIds\":[\"Out1\",\"Out2\"],\"side\":\"RIGHT\"},\"type\":\"ConnectorPlacement.EquallySpacedRectSide\",\"uuid\":\"f7aac5c9-4e6b-4b0b-a99e-124a22eab803\"},{\"content\":{\"side\":\"TOP\"},\"type\":\"ConnectorPlacement.EquallySpacedRectSide\",\"uuid\":\"791bb2d5-f4db-46e5-b405-e7e666275d8b\"},{\"content\":{\"connectorIds\":[\"Out3\"],\"side\":\"BOTTOM\"},\"type\":\"ConnectorPlacement.EquallySpacedRectSide\",\"uuid\":\"b0b7b589-8650-446a-b530-e4865644ee8e\"}]},\"type\":\"ConnectorPlacement.EquallySpacedConnector\",\"uuid\":\"fa79ae73-0718-4a11-9c0b-03878e9e1adb\"}],\"packageUris\":[\"http://schema.mathworks.com/mf0/Connector/R2020b\"],\"version\":\"1.0\"}"
  MATLAB Function1 : MATLAB Function  TreatAsAtomicUnit=on
  α : Outport
  β : Outport  Port=2
  wires:
  target/1 -> MATLAB Function1/1(real)
  MATLAB Function1/1(y) -> Clark1/1(abc)
  Clark1/2(β) -> β/1
  Clark1/1(α) -> α/1
  ICB/1 -> Clark1/2(B)

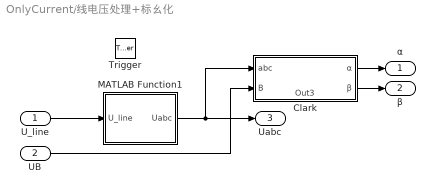
== system OnlyCurrent/线电压处理+标幺化 ==
  U_line : Inport  LatchByDelayingOutsideSignal=on
  UB : Inport  Port=2
  Trigger : TriggerPort  VariantControl=(inherit)
  Clark : Subsystem  TreatAsAtomicUnit=on
      settings: PortSchema="{\"entries\":[{\"content\":{\"sides\":[{\"content\":{\"connectorIds\":[\"In1\",\"In2\"]},\"type\":\"ConnectorPlacement.EquallySpacedRectSide\",\"uuid\":\"5266b147-56b7-4e2a-a13b-4b3ad7884dce\"},{\"content\":{\"connectorIds\":[\"Out1\",\"Out2\"],\"side\":\"RIGHT\"},\"type\":\"ConnectorPlacement.EquallySpacedRectSide\",\"uuid\":\"f7aac5c9-4e6b-4b0b-a99e-124a22eab803\"},{\"content\":{\"side\":\"TOP\"},\"type\":\"ConnectorPlacement.EquallySpacedRectSide\",\"uuid\":\"791bb2d5-f4db-46e5-b405-e7e666275d8b\"},{\"content\":{\"connectorIds\":[\"Out3\"],\"side\":\"BOTTOM\"},\"type\":\"ConnectorPlacement.EquallySpacedRectSide\",\"uuid\":\"b0b7b589-8650-446a-b530-e4865644ee8e\"}]},\"type\":\"ConnectorPlacement.EquallySpacedConnector\",\"uuid\":\"fa79ae73-0718-4a11-9c0b-03878e9e1adb\"}],\"packageUris\":[\"http://schema.mathworks.com/mf0/Connector/R2020b\"],\"version\":\"1.0\"}"
  MATLAB Function1 : MATLAB Function  TreatAsAtomicUnit=on
  α : Outport
  β : Outport  Port=2
  Uabc : Outport  Port=3
  wires:
  U_line/1 -> MATLAB Function1/1(U_line)
  MATLAB Function1/1(Uabc) -> Clark/1(abc), Uabc/1
  Clark/1(α) -> α/1
  Clark/2(β) -> β/1
  UB/1 -> Clark/2(B)

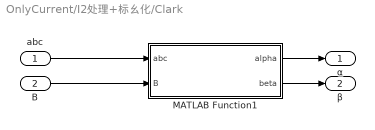
== system OnlyCurrent/I2处理+标幺化/Clark ==
  abc : Inport
  B : Inport  Port=2
  MATLAB Function1 : MATLAB Function  TreatAsAtomicUnit=on
  α : Outport
  β : Outport  Port=2
  wires:
  MATLAB Function1/1(alpha) -> α/1
  abc/1 -> MATLAB Function1/1(abc)
  MATLAB Function1/2(beta) -> β/1
  B/1 -> MATLAB Function1/2(B)

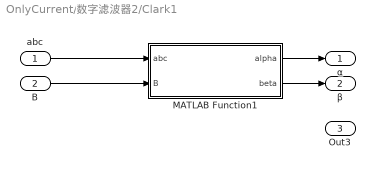
== system OnlyCurrent/数字滤波器2/Clark1 ==
  abc : Inport
  B : Inport  Port=2
  MATLAB Function1 : MATLAB Function  TreatAsAtomicUnit=on
  α : Outport
  β : Outport  Port=2
  Out3 : Outport  Port=3
  wires:
  MATLAB Function1/1(alpha) -> α/1
  abc/1 -> MATLAB Function1/1(abc)
  MATLAB Function1/2(beta) -> β/1
  B/1 -> MATLAB Function1/2(B)

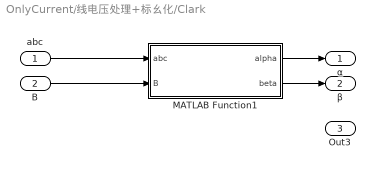
== system OnlyCurrent/线电压处理+标幺化/Clark ==
  abc : Inport
  B : Inport  Port=2
  MATLAB Function1 : MATLAB Function  TreatAsAtomicUnit=on
  α : Outport
  β : Outport  Port=2
  Out3 : Outport  Port=3
  wires:
  MATLAB Function1/1(alpha) -> α/1
  abc/1 -> MATLAB Function1/1(abc)
  MATLAB Function1/2(beta) -> β/1
  B/1 -> MATLAB Function1/2(B)

== matlab function OnlyCurrent/Triggered Subsystem1/MATLAB Function1 ==
  settings: updateMethod=DISCRETE
  data: e input; u_r_prev1 input; u_r_prev2 input; e_prev1 input; e_prev2 input; Kp input; Kr input; wc input; w0 input; u_out output; u_r_state output; Ts input
function [u_out, u_r_state] = QPR_Controller(e, u_r_prev1, u_r_prev2, e_prev1, e_prev2, Kp, Kr, wc, w0, Ts)
% QPR电流环控制器（离散化实现，Tustin变换）
% 输入：
%   e         : 当前时刻电流误差 (i_ref - i_meas)
%   u_r_prev1 : 谐振项上一时刻输出 u_r(k-1)
%   u_r_prev2 : 谐振项上上时刻输出 u_r(k-2)
%   e_prev1   : 上一时刻误差 e(k-1)
%   e_prev2   : 上上时刻误差 e(k-2)
%   Kp, Kr    : 比例系数、谐振系数
%   wc        : 截止频率 (rad/s)
%   w0        : 谐振频率 (rad/s)，如 2*pi*50
%   Ts        : 采样周期 (s)
%
% 输出：
%   u_out     : QPR控制器输出
%   u_r_state : 谐振项当前输出（用于下一时刻状态更新）

% 计算离散化系数
xi = 2 * wc;
den = 4 + 2*xi*Ts + w0^2*Ts^2;

a1 = 2 * (w0^2*Ts^2 - 4) / den;
a2 = (4 - 2*xi*Ts + w0^2*Ts^2) / den;
b0 = 4 * Kr * xi * Ts / den;
b1 = 0;
b2 = -b0;

% 谐振项差分方程迭代
u_r = b0*e + b1*e_prev1 + b2*e_prev2 - a1*u_r_prev1 - a2*u_r_prev2;

% 比例项 + 谐振项
u_out = Kp * e + u_r;

% 输出当前谐振项状态（供下一周期使用）
u_r_state = u_r;
end

== matlab function OnlyCurrent/α,β转SVPWM调制波/MATLAB Function1 ==
  settings: updateMethod=DISCRETE
  data: valpha_pu input; A_SVM output; B_SVM output; vbeta_pu input; C_SVM output; Vbase input; Udc input
function [A_SVM, B_SVM, C_SVM] = ...
    svpwm_simple_pu(valpha_pu, vbeta_pu, Vbase, Udc)
%#codegen

% 母线电压尚未建立时，输出零线电压指令
if Udc <= 1e-6
    A_SVM = 0.5;
    B_SVM = 0.5;
    C_SVM = 0.5;
    return;
end

% 将控制器输出恢复为实际电压
Va = valpha_pu * Vbase;
Vb = vbeta_pu  * Vbase;

% 反 Clarke 变换
v = [Va, (-Va + sqrt(3)*Vb)/2, ...
         (-Va - sqrt(3)*Vb)/2];

% 超出母线可实现范围时，等比例缩小电压矢量
span = max(v) - min(v);
if span > Udc
    v = v * (Udc / span);
end

% 零序注入，转换为 0～1 上管占空比
v0 = (max(v) + min(v)) / 2;
d = 0.5 + (v - v0) / Udc;
d = min(max(d, 0), 1);

A_SVM = d(1);
B_SVM = d(2);
C_SVM = d(3);
end

== matlab function OnlyCurrent/数字滤波器2/Clark1/MATLAB Function1 ==
  settings: updateMethod=DISCRETE
  data: abc input; alpha output; beta output; B input
function [alpha, beta] = abc2alphabeta_mux(abc, B)
%#codegen
% ABC2ALPHABETA_MUX  输入 mux 后的 3 通道信号，输出 alpha-beta
%   abc : [3 x N] 矩阵，第 1/2/3 行分别为 a/b/c
%   alpha, beta : [1 x N] 行向量（可直接接 Scope / Mux 输出）
%
%   Simulink 用法：
%     Mux (3 inputs) --> MATLAB Function --> 输出 alpha, beta

    % 按行取出三相，兼容 [3x1] 和 [3xN]
    a = abc(1, :);
    b = abc(2, :);
    c = abc(3, :);

    K = 2/3;   % 等幅值 Clarke 系数；改 sqrt(2/3) 为等功率

    alpha = K * ( a - 0.5*b - 0.5*c ) / B;
    beta  = K * ( (sqrt(3)/2) * (b - c) ) / B;
end

== matlab function OnlyCurrent/I2处理+标幺化/MATLAB Function1 ==
  settings: updateMethod=DISCRETE
  data: y output; real input
function y = fcn(real)
   y = real;
end

== matlab function OnlyCurrent/线电压处理+标幺化/MATLAB Function1 ==
  settings: updateMethod=DISCRETE
  data: Uabc output; U_line input
function Uabc = line2phase(U_line)
%#codegen
% 输入 U_line: [Uab; Ubc; Uac]  3x1
% 输出 Uabc : [Ua;  Ub;  Uc ]  3x1

Uab = U_line(1);
Ubc = U_line(2);
Uac = U_line(3);

Ua = ( Uab + Uac) / 3;
Ub = ( Ubc - Uab) / 3;
Uc = -(Ubc + Uac) / 3;

Uabc = [Ua; Ub; Uc];
end

== matlab function OnlyCurrent/数字滤波器2/MATLAB Function1 ==
  settings: updateMethod=DISCRETE
  data: y output; real input
function y = fcn(real)
   y = real;
end

== matlab function OnlyCurrent/θ转α,β/MATLAB Function1 ==
  settings: updateMethod=DISCRETE
  data: theta input; alpha output; beta output
function [alpha, beta] = theta2alphabeta(theta)
%#codegen
% 输入 theta: 电角度 (rad)
% 输出 alpha, beta: αβ 分量

alpha = cos(theta);
beta  = sin(theta);

end

== matlab function OnlyCurrent/线电压处理+标幺化/Clark/MATLAB Function1 ==
  settings: updateMethod=DISCRETE
  data: abc input; alpha output; beta output; B input
function [alpha, beta] = abc2alphabeta_mux(abc, B)
%#codegen
% ABC2ALPHABETA_MUX  输入 mux 后的 3 通道信号，输出 alpha-beta
%   abc : [3 x N] 矩阵，第 1/2/3 行分别为 a/b/c
%   alpha, beta : [1 x N] 行向量（可直接接 Scope / Mux 输出）
%
%   Simulink 用法：
%     Mux (3 inputs) --> MATLAB Function --> 输出 alpha, beta

    % 按行取出三相，兼容 [3x1] 和 [3xN]
    a = abc(1, :);
    b = abc(2, :);
    c = abc(3, :);

    K = 2/3;   % 等幅值 Clarke 系数；改 sqrt(2/3) 为等功率

    alpha = K * ( a - 0.5*b - 0.5*c ) / B;
    beta  = K * ( (sqrt(3)/2) * (b - c) ) / B;
end

== matlab function OnlyCurrent/SOGI-FLL Subsystem3/MATLAB Function1 ==
  settings: updateMethod=DISCRETE
  data: u input; theta output; omega output; Ts input
function [theta, omega] = DSOGI_FLL(u, Ts)
% DSOGI-FLL (输入为Mux后的三相电压向量)
% 输入:
%   u  - 3x1 向量 [Ua; Ub; Uc]
%   Ts - 采样周期 (全局变量, 从工作区传入)
% 输出:
%   theta - 估计相角 (rad)
%   omega - 估计角频率 (rad/s)

% --- 持久变量 (状态) ---
persistent x1_alpha x2_alpha x1_beta x2_beta omega_est
if isempty(x1_alpha)
    x1_alpha = 0; x2_alpha = 0;
    x1_beta  = 0; x2_beta  = 0;
    omega_est = 2*pi*50;   % 初始频率 50 Hz
end

% --- 参数 ---
k      = sqrt(2);        % SOGI 增益
Gamma  = 100;            % FLL 增益
omega_n = 2*pi*50;       % 额定角频率

% --- 1) Clarke 变换 (等幅值) ---
Ua = u(1);  Ub = u(2);  Uc = u(3);
ualpha = (2/3) * (Ua - 0.5*Ub - 0.5*Uc);
ubeta  = (2/3) * ( (sqrt(3)/2)*Ub - (sqrt(3)/2)*Uc );

% --- 2) 限幅保护 ---
omega_est = max(min(omega_est, 2*pi*65), 2*pi*45);

% --- 3) SOGI 离散化 (后向欧拉) ---
% alpha 轴
err_a  = ualpha - x1_alpha;
x1_alpha = x1_alpha + Ts * (k * err_a - x2_alpha) * omega_est;
x2_alpha = x2_alpha + Ts * (x1_alpha * omega_est);

% beta 轴
err_b  = ubeta - x1_beta;
x1_beta = x1_beta + Ts * (k * err_b - x2_beta) * omega_est;
x2_beta = x2_beta + Ts * (x1_beta * omega_est);

% --- 4) 正序分量 (Lyon变换简化形式) ---
v_alpha_pos = 0.5 * (x1_alpha - x2_beta);
v_beta_pos  = 0.5 * (x1_beta  + x2_alpha);

% --- 5) FLL 频率估计 ---
epsilon_f = v_alpha_pos * (x1_beta - ubeta) - v_beta_pos * (x1_alpha - ualpha);

% 归一化 (使 Gamma 与电压幅值无关)
norm_factor = v_alpha_pos^2 + v_beta_pos^2;
if norm_factor > 1e-6
    epsilon_f = epsilon_f / norm_factor;
end

omega_est = omega_est - Gamma * epsilon_f * Ts;

% --- 6) 相角输出 ---
theta = atan2(v_beta_pos, v_alpha_pos);
omega = omega_est;

end

== matlab function OnlyCurrent/Triggered Subsystem4/MATLAB Function1 ==
  settings: updateMethod=DISCRETE
  data: e input; u_r_prev1 input; u_r_prev2 input; e_prev1 input; e_prev2 input; Kp input; Kr input; wc input; w0 input; u_out output; u_r_state output; Ts input
function [u_out, u_r_state] = QPR_Controller(e, u_r_prev1, u_r_prev2, e_prev1, e_prev2, Kp, Kr, wc, w0, Ts)
% QPR电流环控制器（离散化实现，Tustin变换）
% 输入：
%   e         : 当前时刻电流误差 (i_ref - i_meas)
%   u_r_prev1 : 谐振项上一时刻输出 u_r(k-1)
%   u_r_prev2 : 谐振项上上时刻输出 u_r(k-2)
%   e_prev1   : 上一时刻误差 e(k-1)
%   e_prev2   : 上上时刻误差 e(k-2)
%   Kp, Kr    : 比例系数、谐振系数
%   wc        : 截止频率 (rad/s)
%   w0        : 谐振频率 (rad/s)，如 2*pi*50
%   Ts        : 采样周期 (s)
%
% 输出：
%   u_out     : QPR控制器输出
%   u_r_state : 谐振项当前输出（用于下一时刻状态更新）

% 计算离散化系数
xi = 2 * wc;
den = 4 + 2*xi*Ts + w0^2*Ts^2;

a1 = 2 * (w0^2*Ts^2 - 4) / den;
a2 = (4 - 2*xi*Ts + w0^2*Ts^2) / den;
b0 = 4 * Kr * xi * Ts / den;
b1 = 0;
b2 = -b0;

% 谐振项差分方程迭代
u_r = b0*e + b1*e_prev1 + b2*e_prev2 - a1*u_r_prev1 - a2*u_r_prev2;

% 比例项 + 谐振项
u_out = Kp * e + u_r;

% 输出当前谐振项状态（供下一周期使用）
u_r_state = u_r;
end

== matlab function OnlyCurrent/I2处理+标幺化/Clark/MATLAB Function1 ==
  settings: updateMethod=DISCRETE
  data: abc input; alpha output; beta output; B input
function [alpha, beta] = abc2alphabeta_mux(abc, B)
%#codegen
% ABC2ALPHABETA_MUX  输入 mux 后的 3 通道信号，输出 alpha-beta
%   abc : [3 x N] 矩阵，第 1/2/3 行分别为 a/b/c
%   alpha, beta : [1 x N] 行向量（可直接接 Scope / Mux 输出）
%
%   Simulink 用法：
%     Mux (3 inputs) --> MATLAB Function --> 输出 alpha, beta

    % 按行取出三相，兼容 [3x1] 和 [3xN]
    a = abc(1, :);
    b = abc(2, :);
    c = abc(3, :);

    K = 2/3;   % 等幅值 Clarke 系数；改 sqrt(2/3) 为等功率

    alpha = K * ( a - 0.5*b - 0.5*c ) / B;
    beta  = K * ( (sqrt(3)/2) * (b - c) ) / B;
end
